simulink model "bess_fcr_twin"  (R2025a)
settings: Solver=ode23t  StartTime=0.0  StopTime=stop_time  MaxStep=0.1  RelTol=1e-7
values from neighbouring files (symbols this model uses):
  caps = m.caps_mw(:)'    [run_twin.m]
  p_base = 0    [run_twin.m]
libraries: nesl_utility x4, fl_lib x3, batteryecm_lib x1, simulink x1
settings Model: Creator=marce  LastModifiedBy=marce
settings DataIOCC: SaveOutput=off  SaveTime=off

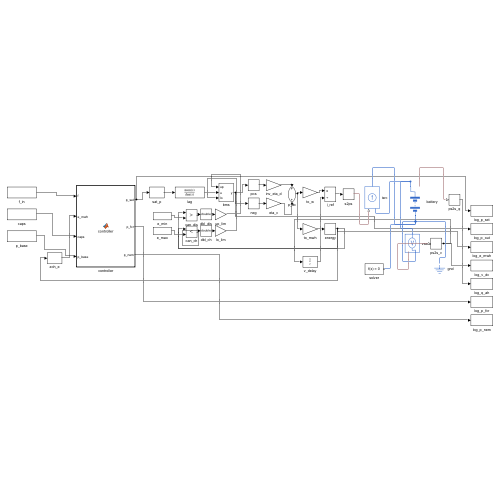
[thumbnail: Simulink's stored preview of the top-level diagram]
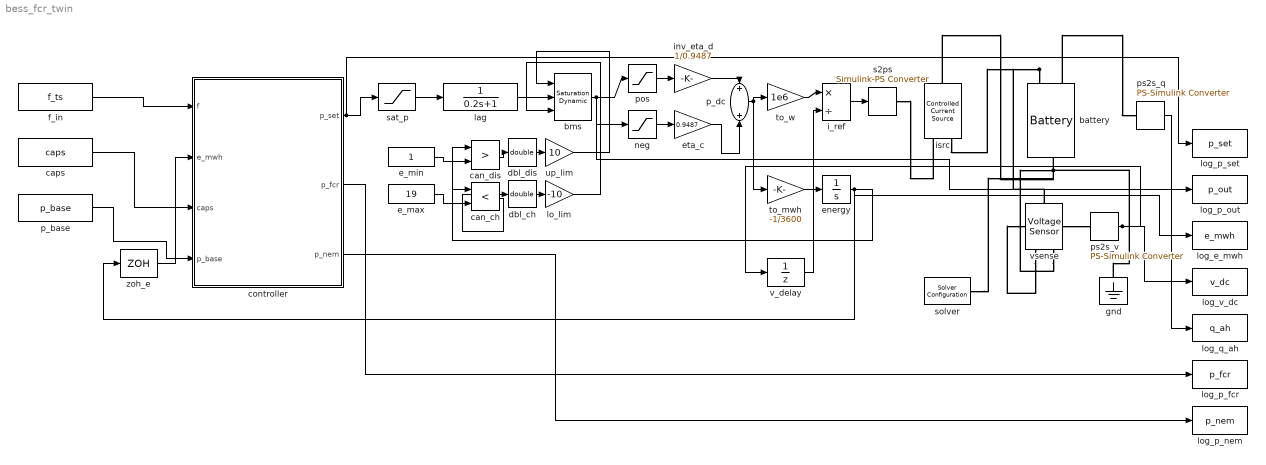
== system bess_fcr_twin ==
  battery : batteryecm_lib/Battery  Vnom=1200 V  prm_dir=simscape.enum.battery.prm_dir.disabled  R1_dis=2 Ohm  R1_ch=2 Ohm  R1=0.0005 Ohm  prm_AH=simscape.enum.battery.prm_AH.finite  AH=16666.6667 A*hr  V1=1176 V  AH1=8333.3333 A*hr  prm_R2=simscape.enum.battery.prm_R2.disabled  R2=2000 Ohm  Tmeas=298.15 K  charge_measurement_port=simscape.enum.battery.enable.yes  prm_dyn=simscape.enum.battery.prm_dyn.off  Rp1=0.005 Ohm  tau1=30 s  Rp2=0.005 Ohm  tau2=30 s  Rp3=0.005 Ohm  tau3=30 s  Rp4=0.005 Ohm  tau4=30 s  Rp5=0.005 Ohm  tau5=30 s  prm_fade=simscape.enum.battery.prm_fade.disabled  N_fade=100  AH_fade=45 A*hr  R1_fade=2.02 Ohm  R1_ch_fade=2.02 Ohm  V1_fade=10.35 V  prm_age=simscape.enum.battery.prm_age.disabled  prm_age_OCV=simscape.enum.battery.prm_age_OCV.OCV  OCV_age=0.9  SOC_age=60  Tmeas_age=298.15 K  delta_time_age_vec=[0] d  temperature_age_vec=[273] K  OCV_scaling_age=2.2134e6  OCV_offset_age=1.632e6  temp_exp_age=0.515833569 V  t_exp_age=0.75  Vnom_T2=12 V  R1_T2=2.2 Ohm  R1_T2_dis=2.2 Ohm  R1_T2_ch=2.2 Ohm  V1_T2=11.4 V  R2_T2=2200 Ohm  Rp1_T2=0.005 Ohm  tau1_T2=30 s  Rp2_T2=0.005 Ohm  tau2_T2=30 s  Rp3_T2=0.005 Ohm  tau3_T2=30 s  Rp4_T2=0.005 Ohm  tau4_T2=30 s  Rp5_T2=0.005 Ohm  tau5_T2=30 s  Tmeas2=273.15 K  thermal_port=simscape.enum.thermaleffects.omit  thermal_mass=30000 J/K  i_specify=off  i_priority=None  i=0 A  i_nominal_specify=off  i_nominal_value=1  i_nominal_unit=A  v_specify=off  v_priority=None  v=0 V  v_nominal_specify=off  v_nominal_value=1  v_nominal_unit=V  charge_specify=on  charge_priority=High  charge=8333.3333 A*hr  charge_nominal_specify=off  charge_nominal_value=1  charge_nominal_unit=A*hr  num_cycles_specify=off  num_cycles_priority=High  num_cycles=0  num_cycles_nominal_specify=off  num_cycles_nominal_value=1  num_cycles_nominal_unit=1  temperature_specify=off  temperature_priority=High  temperature=298.15 K  temperature_nominal_specify=off  temperature_nominal_value=1  temperature_nominal_unit=K
      settings: InternalSimscapePortConfiguration="{\"Bottom\":[],\"Left\":[{\"id\":\"p\",\"label\":\"+\",\"type\":\"foundation.electrical.electrical\"},{\"id\":\"q\",\"label\":\"q\",\"type\":\"output\"}],\"Right\":[{\"id\":\"n\",\"label\":\"-\",\"type\":\"foundation.electrical.electrical\"}],\"Top\":[]}"
  bms : simulink/Discontinuities/Saturation Dynamic  OutMin=[]  OutMax=[]  OutDataTypeStr=Inherit: Same as second input  OutDataType=fixdt(1, 16)  OutScaling=2^-10  DoSatur=off
  can_ch : RelationalOperator  Operator=<  OutDataTypeStr=boolean  RndMeth=Simplest  InputSameDT=off
  can_dis : RelationalOperator  Operator=>  OutDataTypeStr=boolean  RndMeth=Simplest  InputSameDT=off
  caps : Constant  Value=caps  SampleTime=0.1
  controller : MATLAB Function  TreatAsAtomicUnit=on
  dbl_ch : DataTypeConversion  OutDataTypeStr=double  SaturateOnIntegerOverflow=off  RndMeth=Floor
  dbl_dis : DataTypeConversion  OutDataTypeStr=double  SaturateOnIntegerOverflow=off  RndMeth=Floor
  e_max : Constant  Value=19
  e_min : Constant
  energy : Integrator  InitialCondition=10  LimitOutput=on  UpperSaturationLimit=20  LowerSaturationLimit=0
  eta_c : Gain  Gain=0.9487
  f_in : FromWorkspace  VariableName=f_ts  SampleTime=0.1  Interpolate=off  OutputAfterFinalValue=Holding final value
  gnd : fl_lib/Electrical/Electrical Elements/Electrical Reference
  i_ref : Product  Inputs=*/
  inv_eta_d : Gain  Gain=1/0.9487
  isrc : fl_lib/Electrical/Electrical Sources/Controlled Current Source
  lag : TransferFcn  Numerator=1  Denominator=[0.2 1]
  lo_lim : Gain  Gain=-10
  log_e_mwh : ToWorkspace  VariableName=e_mwh  SaveFormat=Timeseries  SampleTime=0.1
  log_p_fcr : ToWorkspace  VariableName=p_fcr  SaveFormat=Timeseries  SampleTime=0.1
  log_p_nem : ToWorkspace  VariableName=p_nem  SaveFormat=Timeseries  SampleTime=0.1
  log_p_out : ToWorkspace  VariableName=p_out  SaveFormat=Timeseries  SampleTime=0.1
  log_p_set : ToWorkspace  VariableName=p_set  SaveFormat=Timeseries  SampleTime=0.1
  log_q_ah : ToWorkspace  VariableName=q_ah  SaveFormat=Timeseries  SampleTime=0.1
  log_v_dc : ToWorkspace  VariableName=v_dc  SaveFormat=Timeseries  SampleTime=0.1
  neg : Saturate  UpperLimit=0  LowerLimit=-inf
  p_base : Constant  Value=p_base  SampleTime=0.1
  p_dc : Sum
  pos : Saturate  UpperLimit=inf  LowerLimit=0
  ps2s_q : nesl_utility/PS-Simulink Converter  PhysicalDomain=network_engine_domain  SubClassName=ps_output  LeftPortType=input  RightPortType=output  PseudoPeriodic=off  Frequencies=[]  VectorFormat=inherit  Unit=A*hr  AffineConversion=off
  ps2s_v : nesl_utility/PS-Simulink Converter  PhysicalDomain=network_engine_domain  SubClassName=ps_output  LeftPortType=input  RightPortType=output  PseudoPeriodic=off  Frequencies=[]  VectorFormat=inherit  Unit=inherit  AffineConversion=off
  s2ps : nesl_utility/Simulink-PS Converter  PhysicalDomain=network_engine_domain  SubClassName=ps_input  LeftPortType=input  RightPortType=output  PseudoPeriodic=off  Frequencies=[]  NoiseDistribution=none  NoiseParameters=[]  Unit=A  AffineConversion=off  FilteringAndDerivatives=provide  SimscapeFilterOrder=1  InputFilterTimeConstant=0.001  UdotUserProvided=0
  sat_p : Saturate  UpperLimit=10  LowerLimit=-10
  solver : nesl_utility/Solver Configuration  PhysicalDomain=network_engine_domain  SubClassName=solver  LeftPortType=input  RightPortType=generic  Tones=[]  Harmonics=[]  SimulateNoise=off  Profile=off  UseLocalSampling=off  EnableSwitchedLinearOptims=on  FrequencyDomain=off  UseCCode=off  RelTol=0.001  AbsTol=0.001  MinStep=1e-09  ToWorkspace=off  RevertToSquareIcSolve=off  NumHomotopyIterations=100  PhasorMode=off  PhasorModeNumHarmonics=1  ConsistencySolver=NEWTON_XTOL_AFTER_FTOL  IndexReductionMethod=DerivativeReplacement  DoDC=off  ResidualTolerance=1e-09  ConsistencyTolSource=GLOBAL  ConsistencyAbsTol=0.001  ConsistencyRelTol=0.001  ConsistencyTolFactor=0.001  UseLocalSolver=off  LocalSolverChoice=NE_BACKWARD_EULER_ADVANCER  ResolveIndetEquations=on  FunctionEvalNumThread=1  LocalSolverSampleTime=0.001  DoFixedCost=off  MaxNonlinIter=3  MaxModeIter=2  ComputeImpulses=off  ImpulseIterations=2  LinearAlgebra=auto  LinearAlgebraNumThread=0  EquationFormulation=NE_TIME_EF  DelaysMemoryBudget=1024  AutomaticFiltering=on  FilteringTimeConstant=0.001  PartitionStorageMethod=AS_NEEDED  PartitionMemoryBudget=1024  PartitionMethod=ROBUST  MultibodyUseLocalSolver=off  MultibodyLocalSolverChoice=ODE1  MultibodyLocalSolverSampleTime=0.001
  to_mwh : Gain  Gain=-1/3600
  to_w : Gain  Gain=1e6
  up_lim : Gain  Gain=10
  v_delay : UnitDelay  InitialCondition=1200  SampleTime=0.1  HasFrameUpgradeWarning=on
  vsense : fl_lib/Electrical/Electrical Sensors/Voltage Sensor
  zoh_e : ZeroOrderHold  SampleTime=0.1
  wires:
  f_in/1 -> controller/1(f)
  zoh_e/1 -> controller/2(e_mwh)
  caps/1 -> controller/3(caps)
  p_base/1 -> controller/4(p_base)
  controller/1(p_set) -> sat_p/1, log_p_set/1
  sat_p/1 -> lag/1
  lag/1 -> bms/2
  up_lim/1 -> bms/1
  lo_lim/1 -> bms/3
  energy/1 -> can_dis/1, can_ch/1, zoh_e/1, log_e_mwh/1
  e_min/1 -> can_dis/2
  e_max/1 -> can_ch/2
  can_dis/1 -> dbl_dis/1
  dbl_dis/1 -> up_lim/1
  can_ch/1 -> dbl_ch/1
  dbl_ch/1 -> lo_lim/1
  bms/1 -> pos/1, neg/1, log_p_out/1
  pos/1 -> inv_eta_d/1
  neg/1 -> eta_c/1
  inv_eta_d/1 -> p_dc/1
  eta_c/1 -> p_dc/2
  p_dc/1 -> to_mwh/1, to_w/1
  to_mwh/1 -> energy/1
  to_w/1 -> i_ref/1
  v_delay/1 -> i_ref/2
  i_ref/1 -> s2ps/1
  ps2s_v/1 -> v_delay/1, log_v_dc/1
  ps2s_q/1 -> log_q_ah/1
  controller/2(p_fcr) -> log_p_fcr/1
  controller/3(p_nem) -> log_p_nem/1
  connections:
  s2ps/RConn1 -- isrc/RConn1
  isrc/LConn1 -- vsense/RConn2 -- gnd/LConn1 -- battery/RConn1 -- solver/RConn1
  battery/LConn1 -- isrc/RConn2 -- vsense/LConn1
  vsense/RConn1 -- ps2s_v/LConn1
  battery/LConn2 -- ps2s_q/LConn1

== matlab function bess_fcr_twin/controller ==
  data: f input; p_set output; e_mwh input; caps input; p_base input; p_fcr output; p_nem output; P parameter
function [p_set, p_fcr, p_nem] = controller(f, e_mwh, caps, p_base, P)
%#codegen
% Mirrors nordic_bess.sim.engine with nordic_bess.control (FCR v1.1, eq. 12-26).
persistent state
if isempty(state)
    state = fcr_controller_init(P);
end
[p_set, state, p_fcr, p_nem] = fcr_controller_step(f, e_mwh, caps, p_base, state, P);
